simulink model "s_c_nbe_m1k"  (R2016b)
settings: Solver=VariableStepAuto  StartTime=0.0  StopTime=1000  RelTol=1e-3  EnableMultiTasking=on
undefined symbols (not defined in the file): Coeffs, fft_stages, n_taps, output_bits, pfb_coeff_gen_calc, xengbits
libraries: xbsIndex_r4 x23639, casper_library_misc x65, casper_library_scopes x4, xbsReplacements_r4 x4, xps_library x3
(part 45 of 198)

== system s_c_nbe_m1k/hmc_ct/gen_freq_calc ==
  note: xengine on board
  note: board
  sync : Inport
  dv : Inport  Port=2
  freq_offset : Inport  Port=3
  AddSub{,3..4,6} (4 alike) : xbsIndex_r4/AddSub  mode=Addition  use_carryin=off  use_carryout=off  en=off  latency=lat  precision=User Defined  arith_type=Unsigned  n_bits=fft_stages-1  bin_pt=0  quantization=Truncate  overflow=Wrap  use_behavioral_HDL=on  hw_selection=Fabric  pipelined=off  dbl_ovrd=off  block_type=addsub
  AddSub1 : xbsIndex_r4/AddSub  mode=Subtraction  use_carryin=off  use_carryout=off  en=off  latency=lat  precision=User Defined  arith_type=Unsigned  n_bits=max_x_per_board_bits  bin_pt=0  quantization=Truncate  overflow=Wrap  use_behavioral_HDL=on  hw_selection=Fabric  pipelined=off  dbl_ovrd=off  block_type=addsub
  AddSub2 : xbsIndex_r4/AddSub  mode=Subtraction  use_carryin=off  use_carryout=off  en=off  latency=lat  precision=User Defined  arith_type=Unsigned  n_bits=max_x_boards_bits  bin_pt=0  quantization=Truncate  overflow=Wrap  use_behavioral_HDL=on  hw_selection=Fabric  pipelined=off  dbl_ovrd=off  block_type=addsub
  Concat1 : xbsIndex_r4/Concat  num_inputs=2  dbl_ovrd=off  block_type=concat
  Constant : xbsIndex_r4/Constant  const=16  gui_display_data_type=Fixed-point  arith_type=Unsigned  n_bits=5  bin_pt=0  preci_type=Single  exp_width=8  frac_width=24  explicit_period=on  period=1  equ=P=C  opselect=C  inp2=PCIN>>17  opr=+  inp1=P  carry=CIN  dbl_ovrd=off  block_type=constant
  Constant1 : xbsIndex_r4/Constant  const=0  gui_display_data_type=Fixed-point  arith_type=Unsigned  n_bits=4  bin_pt=0  preci_type=Single  exp_width=8  frac_width=24  explicit_period=off  period=1  equ=P=C  opselect=C  inp2=PCIN>>17  opr=+  inp1=P  carry=CIN  dbl_ovrd=off  block_type=constant
  Constant2 : xbsIndex_r4/Constant  const=8  gui_display_data_type=Fixed-point  arith_type=Unsigned  n_bits=4  bin_pt=0  preci_type=Single  exp_width=8  frac_width=24  explicit_period=on  period=1  equ=P=C  opselect=C  inp2=PCIN>>17  opr=+  inp1=P  carry=CIN  dbl_ovrd=off  block_type=constant
  Constant3 : xbsIndex_r4/Constant  const=4  gui_display_data_type=Fixed-point  arith_type=Unsigned  n_bits=3  bin_pt=0  preci_type=Single  exp_width=8  frac_width=24  explicit_period=on  period=1  equ=P=C  opselect=C  inp2=PCIN>>17  opr=+  inp1=P  carry=CIN  dbl_ovrd=off  block_type=constant
  Delay{,1..29,32..42} (41 alike) : xbsIndex_r4/Delay  rst=off  infoeditControl=Selection of Reset will increase slice count due to use of real FFs and instead of SRLs  en=off  latency=lat  reg_retiming=on  dbl_ovrd=off  block_type=delay
      settings: infoedit=Hardware notes: A delay line is a chain, each link of which is an SRL16 or SRL32 followed by a flip-flop.
  Gateway Out{1..24} (24 alike) : xbsIndex_r4/Gateway Out  inherit_from_input=off  hdl_port=off  rows=1  columns=1  UseAsDAC=off  DACChannel='1'  interface=None  automatic_assignment=on  address_offset=hex2dec('00')  intf_name=''  intf_description=''  timing_constraint=None  locs_specified=off  LOCs={}  io_standard={}  block_type=gatewayout
  Logical : xbsIndex_r4/Logical  logical_function=OR  inputs=2  en=off  latency=0  precision=Full  arith_type=Unsigned  n_bits=16  bin_pt=0  align_bp=on  dbl_ovrd=off  block_type=logical
  Mult : xbsIndex_r4/Mult  precision=User Defined  arith_type=Unsigned  n_bits=fft_stages - 1 - 2 - 2  bin_pt=0  quantization=Truncate  overflow=Wrap  en=off  latency=lat  use_behavioral_HDL=on  opt=Speed  use_embedded=on  optimum_pipeline=off  pipeline=on  dbl_ovrd=off  use_rpm=on  placement_style=Triangular  block_type=mult
  Mult1 : xbsIndex_r4/Mult  precision=User Defined  arith_type=Unsigned  n_bits=fft_stages-1-2-2  bin_pt=0  quantization=Truncate  overflow=Wrap  en=off  latency=lat  use_behavioral_HDL=on  opt=Speed  use_embedded=on  optimum_pipeline=off  pipeline=on  dbl_ovrd=off  use_rpm=on  placement_style=Triangular  block_type=mult
  Mult2 : xbsIndex_r4/Mult  precision=User Defined  arith_type=Unsigned  n_bits=fft_stages - 1 - 2 - 1  bin_pt=0  quantization=Truncate  overflow=Wrap  en=off  latency=lat  use_behavioral_HDL=on  opt=Speed  use_embedded=on  optimum_pipeline=off  pipeline=on  dbl_ovrd=off  use_rpm=on  placement_style=Triangular  block_type=mult
  Mult3 : xbsIndex_r4/Mult  precision=User Defined  arith_type=Unsigned  n_bits=max_x_boards_bits+max_x_per_board_bits  bin_pt=0  quantization=Truncate  overflow=Wrap  en=off  latency=lat  use_behavioral_HDL=on  opt=Speed  use_embedded=on  optimum_pipeline=off  pipeline=on  dbl_ovrd=off  use_rpm=on  placement_style=Triangular  block_type=mult
  Mult4 : xbsIndex_r4/Mult  precision=User Defined  arith_type=Unsigned  n_bits=max_x_per_board_bits+max_x_boards_bits  bin_pt=0  quantization=Truncate  overflow=Wrap  en=off  latency=lat  use_behavioral_HDL=on  opt=Speed  use_embedded=on  optimum_pipeline=off  pipeline=on  dbl_ovrd=off  use_rpm=on  placement_style=Triangular  block_type=mult
  Mult5 : xbsIndex_r4/Mult  precision=User Defined  arith_type=Unsigned  n_bits=max_x_boards_bits  bin_pt=0  quantization=Truncate  overflow=Wrap  en=off  latency=3  use_behavioral_HDL=on  opt=Speed  use_embedded=on  optimum_pipeline=off  pipeline=on  dbl_ovrd=off  use_rpm=on  placement_style=Triangular  block_type=mult
  Mult6 : xbsIndex_r4/Mult  precision=User Defined  arith_type=Unsigned  n_bits=fft_stages-1  bin_pt=0  quantization=Truncate  overflow=Wrap  en=off  latency=lat  use_behavioral_HDL=on  opt=Speed  use_embedded=on  optimum_pipeline=off  pipeline=on  dbl_ovrd=off  use_rpm=on  placement_style=Triangular  block_type=mult
  Mult7 : xbsIndex_r4/Mult  precision=User Defined  arith_type=Unsigned  n_bits=fft_stages-1  bin_pt=0  quantization=Truncate  overflow=Wrap  en=off  latency=lat  use_behavioral_HDL=on  opt=Speed  use_embedded=on  optimum_pipeline=off  pipeline=on  dbl_ovrd=off  use_rpm=on  placement_style=Triangular  block_type=mult
  Mux : xbsIndex_r4/Mux  inputs=2  en=off  latency=lat  precision=Full  arith_type=Unsigned  n_bits=16  bin_pt=14  quantization=Truncate  overflow=Wrap  dbl_ovrd=off  block_type=mux
  Mux1 : xbsIndex_r4/Mux  inputs=2  en=off  latency=lat  precision=Full  arith_type=Unsigned  n_bits=16  bin_pt=14  quantization=Truncate  overflow=Wrap  dbl_ovrd=off  block_type=mux
  Mux2 : xbsIndex_r4/Mux  inputs=2  en=off  latency=lat  precision=Full  arith_type=Unsigned  n_bits=16  bin_pt=14  quantization=Truncate  overflow=Wrap  dbl_ovrd=off  block_type=mux
  Relational : xbsIndex_r4/Relational  mode=a<b  op_type=Bool  en=off  latency=0  dbl_ovrd=off  block_type=relational
  Relational1 : xbsIndex_r4/Relational  mode=a<b  op_type=Bool  en=off  latency=0  dbl_ovrd=off  block_type=relational
  Relational2 : xbsIndex_r4/Relational  mode=a<b  op_type=Bool  en=off  latency=0  dbl_ovrd=off  block_type=relational
  Scope{1..6} (6 alike) : Scope  NumInputPorts=4
  Slice : xbsIndex_r4/Slice  nbits=fft_stages - 1  boolean_output=off  mode=Two Bit Locations  bit1=0  base1=MSB of Input  bit0=pkt_len_bits  base0=LSB of Input  dbl_ovrd=off  block_type=slice
  Slice1 : xbsIndex_r4/Slice  nbits=4  boolean_output=off  mode=Lower Bit Location + Width  bit1=0  base1=MSB of Input  bit0=0  base0=LSB of Input  dbl_ovrd=off  block_type=slice
  Slice2 : xbsIndex_r4/Slice  nbits=pkt_len_bits + fft_stages - 1  boolean_output=off  mode=Lower Bit Location + Width  bit1=0  base1=MSB of Input  bit0=0  base0=LSB of Input  dbl_ovrd=off  block_type=slice
  Slice3 : xbsIndex_r4/Slice  nbits=2  boolean_output=off  mode=Two Bit Locations  bit1=0  base1=MSB of Input  bit0=4  base0=LSB of Input  dbl_ovrd=off  block_type=slice
  Slice4 : xbsIndex_r4/Slice  nbits=pkt_len_bits + fft_stages - 1  boolean_output=off  mode=Lower Bit Location + Width  bit1=0  base1=MSB of Input  bit0=0  base0=LSB of Input  dbl_ovrd=off  block_type=slice
  Slice5 : xbsIndex_r4/Slice  nbits=2  boolean_output=off  mode=Two Bit Locations  bit1=0  base1=MSB of Input  bit0=4  base0=LSB of Input  dbl_ovrd=off  block_type=slice
  Slice6 : xbsIndex_r4/Slice  nbits=fft_stages - 1  boolean_output=off  mode=Two Bit Locations  bit1=0  base1=MSB of Input  bit0=pkt_len_bits  base0=LSB of Input  dbl_ovrd=off  block_type=slice
  Slice7 : xbsIndex_r4/Slice  nbits=3  boolean_output=off  mode=Lower Bit Location + Width  bit1=0  base1=MSB of Input  bit0=0  base0=LSB of Input  dbl_ovrd=off  block_type=slice
  Slice8 : xbsIndex_r4/Slice  nbits=2  boolean_output=off  mode=Lower Bit Location + Width  bit1=0  base1=MSB of Input  bit0=0  base0=LSB of Input  dbl_ovrd=off  block_type=slice
  Slice9 : xbsIndex_r4/Slice  nbits=1  boolean_output=off  mode=Lower Bit Location + Width  bit1=0  base1=MSB of Input  bit0=0  base0=LSB of Input  dbl_ovrd=off  block_type=slice
  freq_ctr : xbsIndex_r4/Counter  cnt_type=Free Running  cnt_to=Inf  operation=Up  start_count=0  cnt_by_val=1  arith_type=Unsigned  n_bits=pkt_len_bits + fft_stages - 1  bin_pt=0  load_pin=on  rst=off  en=on  explicit_period=on  period=1  use_behavioral_HDL=off  implementation=Fabric  dbl_ovrd=off  block_type=counter
  full_ctr : xbsIndex_r4/Counter  cnt_type=Free Running  cnt_to=Inf  operation=Up  start_count=0  cnt_by_val=1  arith_type=Unsigned  n_bits=64  bin_pt=0  load_pin=off  rst=on  en=on  explicit_period=on  period=1  use_behavioral_HDL=off  implementation=Fabric  dbl_ovrd=off  block_type=counter
  raw_ctr64 : Outport
  freq : Outport  Port=2
  x_index : Outport  Port=3
  x_pkt_index : Outport  Port=4
  wires:
  Delay6/1 -> AddSub3/2
  Delay4/1 -> raw_ctr64/1
  Delay3/1 -> freq/1  "FREQ"
  Mult5/1 -> x_index/1  "X_INDEX"
  [ct_chans_per_x_recip] -> Mult5/2
  Delay/1 -> Delay4/1
  Delay5/1 -> Delay/1
  Delay7/1 -> Delay5/1
  Delay10/1 -> Delay7/1
  Delay13/1 -> Delay10/1
  Delay19/1 -> Delay13/1
  freq_ctr/1 -> Slice/1, Gateway Out13/1  "freq"
  Delay18/1 -> Delay12/1
  Mult4/1 -> Delay35/1, AddSub1/2
  Delay14/1 -> AddSub2/1
  AddSub/1 -> Gateway Out20/1, Delay28/1, AddSub4/1
  [ct_chans_per_x] -> Mult6/2
  [ct_x_per_board] -> Mult4/2
  Mult6/1 -> Gateway Out19/1, AddSub/2
  AddSub3/1 -> Delay29/1, AddSub4/2
  AddSub4/1 -> Delay3/1, Gateway Out4/1, Mult5/1
  Mult/1 -> Mult4/1  "ONE"
  [ct_num_xeng_recip] -> Mult/2
  Delay15/1 -> Delay34/1, AddSub1/1
  [ct_chans_per_board] -> Mult7/2
  [ct_num_x_boards] -> Mult3/2
  AddSub1/1 -> Delay39/1, Mult6/1, Delay36/1, Delay27/1  "TWO"
  Delay9/1 -> Gateway Out21/1, Delay6/1
  Slice1/1 -> Delay18/1, Mux/2, Slice7/1  "FOUR"
  Mult7/1 -> AddSub3/1  "THIS"
  AddSub2/1 -> Delay32/1, Mult7/1  "THREE"
  Mult1/1 -> Delay15/1, Mult3/1
  Mult3/1 -> AddSub2/2
  Delay12/1 -> Delay9/1
  sync/1 -> Delay20/1, Gateway Out12/1, Logical/1, full_ctr/1, freq_ctr/1  "IN_synx"
  [ct_num_x_boards_recip] -> Mult1/2
  Slice3/1 -> Gateway Out15/1, Mult/1, Delay17/1, Mult1/1  "GO8"
  Delay17/1 -> Delay14/1
  Logical/1 -> freq_ctr/3
  dv/1 -> Logical/2, full_ctr/2  "IN_dv"
  freq_offset/1 -> Slice2/1
  full_ctr/1 -> Delay19/1, Slice4/1
  Slice/1 -> Slice3/1, Slice1/1  "freq"
  Slice2/1 -> freq_ctr/2
  Constant1/1 -> Concat1/2
  Delay11/1 -> Concat1/1, Gateway Out17/1
  Concat1/1 -> Delay8/1
  Delay16/1 -> Delay11/1
  Slice4/1 -> Slice6/1
  Slice6/1 -> Slice5/1
  Slice5/1 -> Gateway Out14/1, Mult2/1
  [ct_num_xeng_recip] -> Mult2/2
  Mult2/1 -> Delay16/1  "THEEESE"
  Delay8/1 -> AddSub6/1, Gateway Out18/1, AddSub/1
  AddSub6/1 -> Delay1/1
  Delay1/1 -> Delay2/1
  Delay2/1 -> x_pkt_index/1  "NEW_PKT_INDEX"
  Gateway Out12/1 -> Scope3/1
  Gateway Out13/1 -> Scope3/2
  Gateway Out14/1 -> Scope3/3
  Gateway Out15/1 -> Scope3/4
  Gateway Out1/1 -> Scope1/1
  Gateway Out2/1 -> Scope1/2
  Gateway Out3/1 -> Scope1/3
  Gateway Out4/1 -> Scope1/4
  Delay20/1 -> Delay21/1
  Delay21/1 -> Delay22/1
  Delay22/1 -> Delay33/1, Delay23/1
  Delay23/1 -> Delay24/1
  Delay24/1 -> Delay25/1
  Delay25/1 -> Gateway Out1/1
  Gateway Out5/1 -> Scope2/1
  Gateway Out6/1 -> Scope2/2
  Gateway Out7/1 -> Scope2/3
  Gateway Out8/1 -> Scope2/4
  Delay28/1 -> Gateway Out2/1
  Delay29/1 -> Gateway Out3/1
  Delay27/1 -> Gateway Out6/1
  Delay32/1 -> Gateway Out7/1
  Delay33/1 -> Gateway Out5/1
  Gateway Out9/1 -> Scope4/1
  Gateway Out10/1 -> Scope4/2
  Gateway Out11/1 -> Scope4/3
  Gateway Out16/1 -> Scope4/4
  Delay37/1 -> Delay42/1
  Delay38/1 -> Delay41/1
  Delay39/1 -> Delay40/1
  Delay40/1 -> Gateway Out11/1
  Delay41/1 -> Gateway Out10/1
  Delay42/1 -> Gateway Out9/1
  Delay34/1 -> Delay37/1
  Delay35/1 -> Delay38/1
  Delay36/1 -> Gateway Out16/1
  Gateway Out17/1 -> Scope5/1
  Gateway Out18/1 -> Scope5/2
  Gateway Out19/1 -> Scope5/3
  Gateway Out20/1 -> Scope5/4
  Slice7/1 -> Mux/3
  Relational/1 -> Mux/1
  [ct_chans_per_x] -> Relational/1
  Constant/1 -> Relational/2
  Constant2/1 -> Relational1/2
  Relational1/1 -> Mux1/1
  Mux/1 -> Slice8/1, Gateway Out22/1, Mux1/2
  Slice8/1 -> Mux1/3
  Slice9/1 -> Mux2/3
  Mux1/1 -> Gateway Out23/1, Slice9/1, Mux2/2
  [ct_chans_per_x] -> Relational1/1
  Relational2/1 -> Mux2/1
  Constant3/1 -> Relational2/2
  [ct_chans_per_x] -> Relational2/1
  Mux2/1 -> Gateway Out24/1, Delay26/1
  Delay26/1 -> AddSub6/2, Gateway Out8/1
  Gateway Out21/1 -> Scope6/1
  Gateway Out22/1 -> Scope6/2
  Gateway Out24/1 -> Scope6/4
  Gateway Out23/1 -> Scope6/3

== system s_c_nbe_m1k/hmc_ct/hmc_addr_gen ==
  note: Map writes across HMC
      | for performance.
  note: Map the output read to collect like channels.
  note: Read when write switches banks.
  note: Write is linear.
  note: Map writes across HMC
      | for performance.
  sync : Inport
  dv : Inport  Port=2
  d256_0 : Inport  Port=3
  d256_1 : Inport  Port=4
  Concat1 : xbsIndex_r4/Concat  num_inputs=2  dbl_ovrd=off  block_type=concat
  Concat2 : xbsIndex_r4/Concat  num_inputs=2  dbl_ovrd=off  block_type=concat
  Concat3 : xbsIndex_r4/Concat  num_inputs=2  dbl_ovrd=off  block_type=concat
  Constant6 : xbsIndex_r4/Constant  const=0  gui_display_data_type=Fixed-point  arith_type=Unsigned  n_bits=27 - (invec_bits + outvec_bits + 1)  bin_pt=0  preci_type=Single  exp_width=8  frac_width=24  explicit_period=on  period=1  equ=P=C  opselect=C  inp2=PCIN>>17  opr=+  inp1=P  carry=CIN  dbl_ovrd=off  block_type=constant
  Constant8 : xbsIndex_r4/Constant  const=0  gui_display_data_type=Fixed-point  arith_type=Unsigned  n_bits=27 - (invec_bits + outvec_bits + 1)  bin_pt=0  preci_type=Single  exp_width=8  frac_width=24  explicit_period=on  period=1  equ=P=C  opselect=C  inp2=PCIN>>17  opr=+  inp1=P  carry=CIN  dbl_ovrd=off  block_type=constant
  Delay{1..2,4,9,12,18..22} (10 alike) : xbsIndex_r4/Delay  rst=off  infoeditControl=Selection of Reset will increase slice count due to use of real FFs and instead of SRLs  en=off  latency=7*3  reg_retiming=on  dbl_ovrd=off  block_type=delay
      settings: infoedit=Hardware notes: A delay line is a chain, each link of which is an SRL16 or SRL32 followed by a flip-flop.
  Delay{5..8,10,30..35} (11 alike) : xbsIndex_r4/Delay  rst=off  infoeditControl=Selection of Reset will increase slice count due to use of real FFs and instead of SRLs  en=off  latency=1  reg_retiming=on  dbl_ovrd=off  block_type=delay
      settings: infoedit=Hardware notes: A delay line is a chain, each link of which is an SRL16 or SRL32 followed by a flip-flop.
  Delay{3,11,13..16,24..29} (12 alike) : xbsIndex_r4/Delay  rst=off  infoeditControl=Selection of Reset will increase slice count due to use of real FFs and instead of SRLs  en=off  latency=3  reg_retiming=on  dbl_ovrd=off  block_type=delay
      settings: infoedit=Hardware notes: A delay line is a chain, each link of which is an SRL16 or SRL32 followed by a flip-flop.
  Gateway Out{,1..7} (8 alike) : xbsIndex_r4/Gateway Out  inherit_from_input=off  hdl_port=off  rows=1  columns=1  UseAsDAC=off  DACChannel='1'  interface=None  automatic_assignment=on  address_offset=hex2dec('00')  intf_name=''  intf_description=''  timing_constraint=None  locs_specified=off  LOCs={}  io_standard={}  block_type=gatewayout
  Inverter1 : xbsIndex_r4/Inverter  en=off  latency=0  dbl_ovrd=off  block_type=inv
  Scope : Scope  NumInputPorts=4
  Scope1 : Scope  NumInputPorts=4
  Slice : xbsIndex_r4/Slice  nbits=16  boolean_output=off  mode=Upper Bit Location + Width  bit1=0  base1=MSB of Input  bit0=0  base0=LSB of Input  dbl_ovrd=off  block_type=slice
  Slice1 : xbsIndex_r4/Slice  nbits=invec_bits+outvec_bits  boolean_output=off  mode=Lower Bit Location + Width  bit1=0  base1=MSB of Input  bit0=0  base0=LSB of Input  dbl_ovrd=off  block_type=slice
  Slice5 : xbsIndex_r4/Slice  nbits=9  boolean_output=off  mode=Lower Bit Location + Width  bit1=0  base1=MSB of Input  bit0=0  base0=LSB of Input  dbl_ovrd=off  block_type=slice
  bank : xbsIndex_r4/Slice  nbits=1  boolean_output=on  mode=Upper Bit Location + Width  bit1=0  base1=MSB of Input  bit0=0  base0=LSB of Input  dbl_ovrd=off  block_type=slice
  edge_detect2 : Subsystem  AncestorBlock=casper_library_misc/edge_detect  mask(edge_detect){edge=Rising, polarity=Active High, x_in=[0 0.08 0.08 0.16 0.16 0.24 0.24 0.32 0.32 0.4], y_in=[-1 -1  1  1  1  1  1  1  1  1], x_out=[0.6 0.68 0.68 0.76 0.76 0.84 0.84 0.92 0.92 1], y_out=[-1 -1  1  1 -1 -1 -1 -1 -1 -1]}
      mask prompts: edge "Edge Type"; polarity "Output Polarity"; x_in "Input X Positions"; y_in "Input Y Positions"; x_out "Output X Positions"; y_out "Output Y Positions"
      mask help: Output is active for one-cycle after each edge of the specified type (i.e. rising, falling or both).
      mask init: same as s_c_nbe_m1k/edge_detect1
      settings: AttributesFormatString=|
      | rising edges
      | active high
      mask Help: Output is active for one-cycle after each edge of the specified type (i.e. rising, falling, or both).  Latency is zero.
      mask TypeOptions edge: Rising | Falling | Both
      mask TypeOptions polarity: Active High | Active Low
      mask Display:
      | plot(x_in_num,0.5+y_in_num*0.2);
      | plot(x_out_num,0.5+y_out_num*0.2);
  hmc_addr_opt : Subsystem
  hmc_addr_opt1 : Subsystem
  last_tag2 : xbsIndex_r4/Register  init=0  rst=on  en=on  dbl_ovrd=off  block_type=register
  rd_add_ctr : Subsystem
  read_map_calc : Subsystem  mask{rmc_invec_bits=invec_bits, rmc_outvec_bits=outvec_bits, lat=3, max_x_boards_bits=max_x_boards_bits, n_bits_chans_per_word=n_bits_chans_per_word, max_x_per_board_bits=max_x_per_board_bits}
      mask prompts: rmc_invec_bits "Input vector bits"; rmc_outvec_bits "output vector bits"; lat "latency per block"; max_x_boards_bits "max x boards (2^?)"; n_bits_chans_per_word "channels per input word (2^?)"; max_x_per_board_bits "max x engines per board (2^?)"
      mask init:
      | display_string = ['latency=', num2str(lat * 7), '\ninput_vector_bits=', num2str(rmc_invec_bits), '\noutput_vector_bits=', num2str(rmc_outvec_bits)];
      | set_param(gcb, 'AttributesFormatString', display_string);
      settings: AttributesFormatString=latency=21\ninput_vector_bits=6\noutput_vector_bits=8
  waddr : xbsIndex_r4/Counter  cnt_type=Free Running  cnt_to=Inf  operation=Up  start_count=0  cnt_by_val=1  arith_type=Unsigned  n_bits=invec_bits + outvec_bits + 1  bin_pt=0  load_pin=off  rst=on  en=on  explicit_period=on  period=1  use_behavioral_HDL=off  implementation=Fabric  dbl_ovrd=off  block_type=counter
  wr_sync : Outport
  wr_en : Outport  Port=2
  wr_addr : Outport  Port=3
  wr_d256_0 : Outport  Port=4
  wr_d256_1 : Outport  Port=5
  rd_en : Outport  Port=6
  rd_addr : Outport  Port=7
  rd_tag : Outport  Port=8
  rd_addr_arm : Outport  Port=9
  rd_arm_raw : Outport  Port=10
  wires:
  Delay14/1 -> Delay21/1
  Inverter1/1 -> Delay8/1  "IN_bank"
  Delay9/1 -> Gateway Out1/1, [wr_dv]
  Delay18/1 -> Slice/1, [wr_d256_0]
  Delay19/1 -> Gateway Out4/1, [wr_sync]
  Delay16/1 -> Delay2/1  "ZEN_en_input"
  Delay25/1 -> Delay9/1  "ZEN_wr_dv"
  Delay27/1 -> Delay18/1
  Delay28/1 -> Delay19/1
  d256_0/1 -> Delay32/1
  Delay11/1 -> Delay4/1
  Delay29/1 -> Delay20/1
  Concat1/1 -> [rd_addr]
  Delay4/1 -> [rd_addr_arm]  "zen_addr_arm"
  Delay2/1 -> [rd_en], Gateway Out5/1  "zen_rden"
  [rd_now] -> last_tag2/3, last_tag2/1
  Delay1/1 -> [rd_tag]  "zen_rdtag"
  dv/1 -> Delay30/1, rd_add_ctr/2(dv), Delay6/1, waddr/2  "IN_dv"
  waddr/1 -> [wr_addr_cnt], Delay34/1, Slice5/1, Slice1/1, bank/1  "waddr_cnt"
  sync/1 -> Delay35/1, [sync256], waddr/1, rd_add_ctr/1(rd_now), Delay33/1  "IN_sync"
  Delay20/1 -> Gateway Out2/1, hmc_addr_opt/1(addr)  "ZEN_wrctr"
  hmc_addr_opt/1(" addr_opt") -> Concat2/2
  Concat2/1 -> [wr_addr]
  Constant6/1 -> Concat1/1
  Constant8/1 -> Concat2/1
  Delay34/1 -> Delay29/1
  Delay33/1 -> Delay28/1
  Delay32/1 -> Delay27/1
  Delay30/1 -> Delay25/1
  last_tag2/1 -> Delay10/1, [rd_addr_arm_raw]
  [wr_addr] -> wr_addr/1
  [wr_d256_0] -> wr_d256_0/1
  [rd_en] -> rd_en/1
  [rd_addr] -> rd_addr/1
  [rd_tag] -> rd_tag/1
  [wr_sync] -> wr_sync/1
  [rd_addr_arm] -> rd_addr_arm/1
  [rd_addr_arm_raw] -> rd_arm_raw/1
  [wr_dv] -> wr_en/1
  hmc_addr_opt1/1(" addr_opt") -> Concat1/2
  read_map_calc/1(address) -> Concat3/2, Gateway Out6/1  "zen_calc_addr"
  Delay21/1 -> Concat3/1  "zen_bank"
  Delay15/1 -> Delay1/1
  rd_add_ctr/1(rd_ctr) -> Delay13/1
  [ct_board_hmc_offset] -> rd_add_ctr/3(xeng_offset)
  Delay6/1 -> Delay16/1
  Delay8/1 -> Delay14/1
  Delay7/1 -> Delay15/1
  Delay10/1 -> Delay11/1
  Delay13/1 -> read_map_calc/1(raw_address)
  Slice5/1 -> Delay7/1
  [sync256] -> last_tag2/2
  d256_1/1 -> Delay31/1
  Delay26/1 -> Delay12/1
  Delay31/1 -> Delay26/1
  Delay12/1 -> [wr_d256_1]
  [wr_d256_1] -> wr_d256_1/1
  Gateway Out/1 -> Scope/1
  Delay35/1 -> Delay24/1
  Delay24/1 -> Delay22/1
  Gateway Out1/1 -> Scope/2
  Gateway Out2/1 -> Scope/3
  Slice/1 -> Gateway Out3/1
  Gateway Out3/1 -> Scope/4
  Concat3/1 -> Gateway Out7/1, hmc_addr_opt1/1(addr)  "ZEN_wrctr"
  Gateway Out4/1 -> Scope1/1
  Delay22/1 -> Gateway Out/1
  Gateway Out5/1 -> Scope1/2
  Gateway Out6/1 -> Scope1/3
  Gateway Out7/1 -> Scope1/4
  Slice1/1 -> Delay5/1
  bank/1 -> edge_detect2/1(in), Inverter1/1  "wrbank"
  edge_detect2/1(out) -> [rd_now]
  Delay3/1 -> read_map_calc/2(raw_cnt)
  Delay5/1 -> Delay3/1
